simulink model "fft_512_dma"  (R2025b)
settings: Solver=FixedStepDiscrete  StartTime=0.0  StopTime=10.0  RelTol=1e-3
libraries: hdlsllib x4, simulink x1, dsphdlxfrm2 x1
settings Model: DataTypeOverride=Off  Creator=ADMIN  LastModifiedBy=ADMIN
settings OptimizationCC: BlockReduction=off  ConditionallyExecuteInputs=off  DefaultParameterBehavior=Inlined  InheritOutputTypeSmallerThanSingle=on
settings DebuggingCC: ArtificialAlgebraicLoopMsg=error  SingleTaskRateTransMsg=error
settings HardwareCC: ProdBitPerPointer=32.0  ProdBitPerSizeT=32.0  ProdBitPerPtrDiffT=32.0  ProdLargestAtomicFloat=None  ProdIntDivRoundTo=Undefined  ProdEndianess=Unspecified  ProdWordSize=32.0  ProdHWDeviceType=ASIC/FPGA->ASIC/FPGA  TargetBitPerPointer=64.0  TargetBitPerSizeT=64.0  TargetBitPerPtrDiffT=64.0  TargetLongLongMode=on  TargetIntDivRoundTo=Zero  TargetEndianess=LittleEndian  TargetWordSize=64.0  TargetHWDeviceType=Custom Processor->MATLAB Host Computer  ProdEqTarget=off

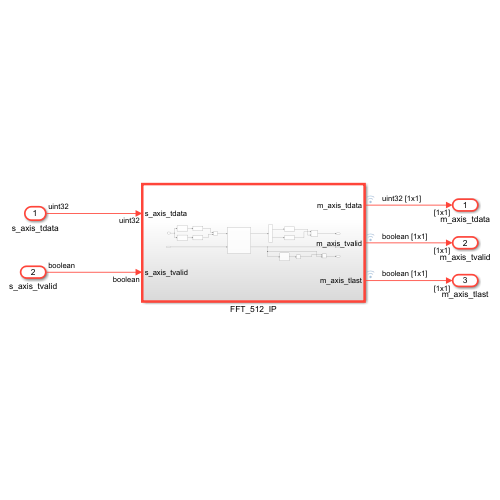
[thumbnail: Simulink's stored preview of the top-level diagram]
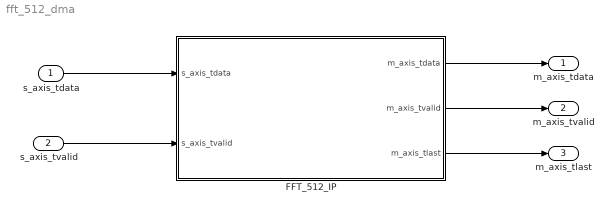
== system fft_512_dma ==
  s_axis_tdata : Inport  OutDataTypeStr=uint32  PortDimensions=1  SampleTime=1
  s_axis_tvalid : Inport  Port=2  OutDataTypeStr=boolean  PortDimensions=1  SampleTime=1
  FFT_512_IP : Subsystem  TreatAsAtomicUnit=on
  m_axis_tdata : Outport
  m_axis_tvalid : Outport  Port=2
  m_axis_tlast : Outport  Port=3
  wires:
  s_axis_tdata/1 -> FFT_512_IP/1(s_axis_tdata)
  s_axis_tvalid/1 -> FFT_512_IP/2(s_axis_tvalid)
  FFT_512_IP/1(m_axis_tdata) -> m_axis_tdata/1
  FFT_512_IP/2(m_axis_tvalid) -> m_axis_tvalid/1
  FFT_512_IP/3(m_axis_tlast) -> m_axis_tlast/1

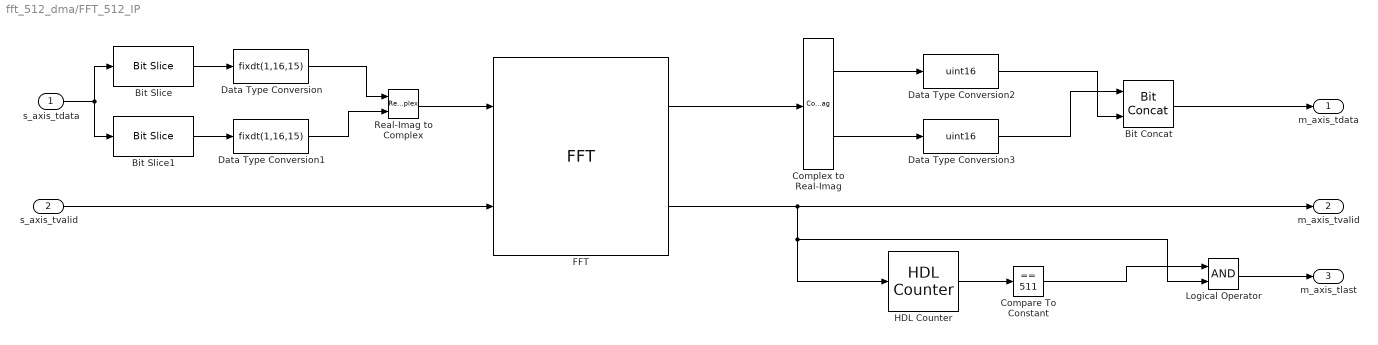
== system fft_512_dma/FFT_512_IP ==
  s_axis_tdata : Inport  OutDataTypeStr=uint32  PortDimensions=1  SampleTime=1
  s_axis_tvalid : Inport  Port=2  OutDataTypeStr=boolean  PortDimensions=1  SampleTime=1
  Bit Concat : hdlsllib/Logic and Bit Operations/Bit Concat  numInputs=2
  Bit Slice : hdlsllib/Logic and Bit Operations/Bit Slice  lidx=15  ridx=0
  Bit Slice1 : hdlsllib/Logic and Bit Operations/Bit Slice  lidx=31  ridx=16
  Compare To Constant : simulink/Logic and Bit Operations/Compare To Constant  relop===  const=511  OutDataTypeStr=boolean
  Complex to Real-Imag : ComplexToRealImag
  Data Type Conversion : DataTypeConversion  OutDataTypeStr=fixdt(1,16,15)  ConvertRealWorld=Stored Integer (SI)  SaturateOnIntegerOverflow=off  RndMeth=Floor
  Data Type Conversion1 : DataTypeConversion  OutDataTypeStr=fixdt(1,16,15)  ConvertRealWorld=Stored Integer (SI)  SaturateOnIntegerOverflow=off  RndMeth=Floor
  Data Type Conversion2 : DataTypeConversion  OutDataTypeStr=uint16  ConvertRealWorld=Stored Integer (SI)  SaturateOnIntegerOverflow=off  RndMeth=Floor
  Data Type Conversion3 : DataTypeConversion  OutDataTypeStr=uint16  ConvertRealWorld=Stored Integer (SI)  SaturateOnIntegerOverflow=off  RndMeth=Floor
  FFT : dsphdlxfrm2/FFT  Architecture=Streaming Radix 2^2  FFTLengthSource=Property  FFTLength=512  FFTLengthMax=1024  ComplexMultiplication=Use 4 multipliers and 2 adders  BitReversedOutput=off  BitReversedInput=off  Normalize=on  SimulateUsing=Code generation  RoundingMethod=Floor  ResetInputPort=off  StartOutputPort=off  EndOutputPort=off
  HDL Counter : hdlsllib/Sources/HDL Counter  CountType=Count limited  CountInit=0  CountStep=1  CountMax=511  CountFromType=Initial value  CountFrom=0  CountResetPort=off  CountLoadPort=off  CountEnbPort=on  CountDirPort=off  CountHitOutputPort=off  CountDataType=Unsigned  CountWordLen=9  CountFracLen=0  CountSampTime=1
  Logical Operator : Logic  AllPortsSameDT=off  OutDataTypeStr=boolean
  Real-Imag to Complex : RealImagToComplex
  m_axis_tdata : Outport
  m_axis_tvalid : Outport  Port=2
  m_axis_tlast : Outport  Port=3
  wires:
  s_axis_tdata/1 -> Bit Slice/1, Bit Slice1/1
  Bit Slice/1 -> Data Type Conversion/1
  Bit Slice1/1 -> Data Type Conversion1/1
  Data Type Conversion/1 -> Real-Imag to Complex/1
  Data Type Conversion1/1 -> Real-Imag to Complex/2
  Real-Imag to Complex/1 -> FFT/1
  s_axis_tvalid/1 -> FFT/2
  Complex to Real-Imag/2 -> Data Type Conversion3/1
  Data Type Conversion3/1 -> Bit Concat/1
  Complex to Real-Imag/1 -> Data Type Conversion2/1
  Data Type Conversion2/1 -> Bit Concat/2
  FFT/1 -> Complex to Real-Imag/1
  Bit Concat/1 -> m_axis_tdata/1
  FFT/2 -> HDL Counter/1, Logical Operator/2, m_axis_tvalid/1
  HDL Counter/1 -> Compare To Constant/1
  Compare To Constant/1 -> Logical Operator/1
  Logical Operator/1 -> m_axis_tlast/1
